simulink model "dcmotor"  (R2016a)
settings: Solver=VariableStepAuto  StartTime=0.0  StopTime=10  RelTol=1e-3
libraries: simulink x1
settings Model: Creator=sanket Pradhan  LastModifiedBy=sanket Pradhan

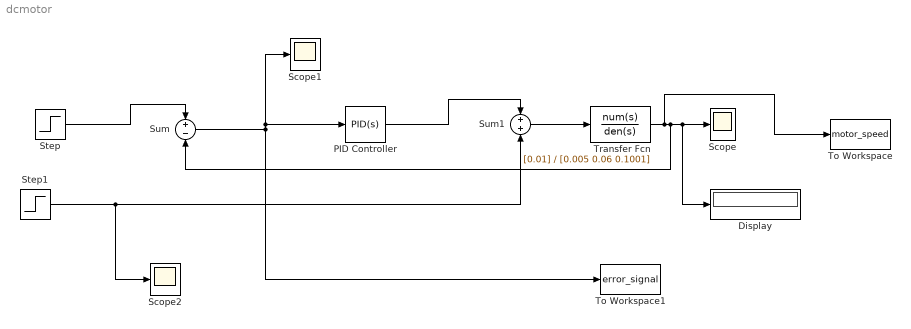
== system dcmotor ==
  Display : Display
  PID Controller : simulink/Continuous/PID Controller  Controller=PID  TimeDomain=Continuous-time  SampleTime=-1  IntegratorMethod=Forward Euler  FilterMethod=Forward Euler  Form=Parallel  UseFilter=on  ControllerParametersSource=internal  P=2  I=4  D=0.1  N=100  InitialConditionSource=internal  InitialConditionForIntegrator=0  InitialConditionForFilter=0  ExternalReset=none  LimitOutput=off  UpperSaturationLimit=inf  LowerSaturationLimit=-inf  LinearizeAsGain=on  AntiWindupMode=none  Kb=1  TrackingMode=off  Kt=1  PParamMin=[]  PParamMax=[]  IParamMin=[]  IParamMax=[]  DParamMin=[]  DParamMax=[]  NParamMin=[]  NParamMax=[]  KbParamMin=[]  KbParamMax=[]  KtParamMin=[]  KtParamMax=[]  POutMin=[]  POutMax=[]  IOutMin=[]  IOutMax=[]  DOutMin=[]  DOutMax=[]  NOutMin=[]  NOutMax=[]  KbOutMin=[]  KbOutMax=[]  KtOutMin=[]  KtOutMax=[]  IntegratorOutMin=[]  IntegratorOutMax=[]  FilterOutMin=[]  FilterOutMax=[]  SumOutMin=[]  SumOutMax=[]  SumI1OutMin=[]  SumI1OutMax=[]  SumI2OutMin=[]  SumI2OutMax=[]  SumI3OutMin=[]  SumI3OutMax=[]  SumDOutMin=[]  SumDOutMax=[]  SaturationOutMin=[]  SaturationOutMax=[]  IntegratorContinuousStateAttributes=''  IntegratorStateMustResolveToSignalObject=off  IntegratorRTWStateStorageClass=Auto  FilterContinuousStateAttributes=''  FilterStateMustResolveToSignalObject=off  FilterRTWStateStorageClass=Auto  DifferentiatorICPrevScaledInput=0  DifferentiatorOutMin=[]  DifferentiatorOutMax=[]
  Scope : Scope
  Scope1 : Scope
  Scope2 : Scope
  Step : Step  Time=0  After=3000  SampleTime=0
  Step1 : Step  Time=5  After=1000  SampleTime=0
  Sum : Sum  Inputs=+-
  Sum1 : Sum
  To Workspace : ToWorkspace  VariableName=motor_speed  SaveFormat=Structure With Time  SampleTime=-1
  To Workspace1 : ToWorkspace  VariableName=error_signal  SaveFormat=Timeseries  SampleTime=-1
  Transfer Fcn : TransferFcn  Numerator=[0.01]  Denominator=[0.005 0.06 0.1001]
  wires:
  Step/1 -> Sum/1
  PID Controller/1 -> Sum1/1
  Transfer Fcn/1 -> Scope/1, Display/1, Sum/2, To Workspace/1
  Sum1/1 -> Transfer Fcn/1
  Sum/1 -> PID Controller/1, Scope1/1, To Workspace1/1
  Step1/1 -> Scope2/1, Sum1/2
